simulink model "Y3Tiltrotor_sim3_IINDI"  (R2025a)
settings: Solver=ode4  StartTime=0.0  StopTime=60  FixedStep=uavParam.sampleTime  RelTol=1e-3
PreLoadFcn:
  | filepath  = fileparts(get_param(bdroot, 'FileName'))
  | cd(filepath);
InitFcn:
  | Init_sim_IINDI;
values from neighbouring files (symbols this model uses):
  a_HOD_p = 5    [Init_sim_IINDI.m]
  a_HOD_q = 5    [Init_sim_IINDI.m]
  a_HOD_r = 5    [Init_sim_IINDI.m]
  a_HOD_u = 5    [Init_sim_IINDI.m]
  a_HOD_v = 2    [Init_sim_IINDI.m]
  a_HOD_w = 30    [Init_sim_IINDI.m]
  control = struct    [Init_sim_IINDI.m]
  env = struct    [InitData.m]
  flightState = struct    [Init_sim_IINDI.m]
  FWSpeed0 = 15    [Init_sim_IINDI.m]
  k_lpf_p = 50    [Init_sim_IINDI.m]
  k_lpf_q = 80    [Init_sim_IINDI.m]
  k_lpf_r = 100    [Init_sim_IINDI.m]
  k_lpf_u = 10    [Init_sim_IINDI.m]
  k_lpf_v = 1.5    [Init_sim_IINDI.m]
  k_lpf_w = 50    [Init_sim_IINDI.m]
  k_p = 5    [Init_sim_IINDI.m]
  k_q = 12    [Init_sim_IINDI.m]
  k_r = 0.1    [Init_sim_IINDI.m]
  k_u = 1    [Init_sim_IINDI.m]
  k_v = 0.7    [Init_sim_IINDI.m]
  k_w = 2    [Init_sim_IINDI.m]
  l_p = 30    [Init_sim_IINDI.m]
  l_q = 15    [Init_sim_IINDI.m]
  l_r = 25    [Init_sim_IINDI.m]
  l_u = 10    [Init_sim_IINDI.m]
  l_v = 1.2    [Init_sim_IINDI.m]
  l_w = 1    [Init_sim_IINDI.m]
  lamda_p = 10    [Init_sim_IINDI.m]
  lamda_q = 5    [Init_sim_IINDI.m]
  lamda_r = 1    [Init_sim_IINDI.m]
  lamda_u = 1    [Init_sim_IINDI.m]
  lamda_v = 0.15    [Init_sim_IINDI.m]
  lamda_w = 1    [Init_sim_IINDI.m]
  uavParam = struct    [InitData.m]
undefined symbols (not defined in the file or in its folder): a_HOD, a_HOD_uvw, ControlSampleTime, F, Light, MIL, Newton, Raphson
libraries: slpidlib x30, SignalEditorBlockLib x13, simulink x3, aerolibtransform2 x3, sharedtransform x3, robotcorelib x3, matrix_library x3, aerolibasang x2, aerolibutil x2, aerolibwind2 x2, shared6dof x1, aerolibatmos2 x1
(part 5 of 7)

== system Y3Tiltrotor_sim3_IINDI/Subsystem/固定翼模态/高度-速度控制/定速模式/airspeed control ==
  Manual : Inport
  Airspeed_d : Inport  Port=2
  V_ref : Inport  Port=3
  Airspeed : Inport  Port=4
  PID Controller1 : slpidlib/PID Controller  Controller=PID  Form=Parallel  TimeDomain=Continuous-time  UseExternalTs=off  SampleTime=ControlSampleTime  IntegratorMethod=Forward Euler  FilterMethod=Forward Euler  ControllerParametersSource=internal  P=control.FW.airspeed_P  I=control.FW.airspeed_I  UseKiTs=off  D=control.FW.airspeed_D  UseExternalDerivativeSource=off  N=100  UseFilter=on  TunerSelectOption=Transfer Function Based (PID Tuner App)  InitialConditionSource=internal  InitialConditionForIntegrator=0  InitialConditionForFilter=0  DifferentiatorICPrevScaledInput=0  ExternalReset=none  TrackingMode=off  Kt=1  LimitOutput=on  SatLimitsSource=internal  UpperSaturationLimit=1  LowerSaturationLimit=0  LinearizeAsGain=on  AntiWindupMode=clamping  Kb=1  LimitIntegrator=off  UpperIntegratorSaturationLimit=inf  LowerIntegratorSaturationLimit=-inf  POutMin=[]  POutMax=[]  IOutMin=[]  IOutMax=[]  DOutMin=[]  DOutMax=[]  NOutMin=[]  NOutMax=[]  SumOutMin=[]  SumOutMax=[]  SaturationOutMin=[]  SaturationOutMax=[]  PParamMin=[]  PParamMax=[]  IParamMin=[]  IParamMax=[]  DParamMin=[]  DParamMax=[]  NParamMin=[]  NParamMax=[]  KbParamMin=[]  KbParamMax=[]  KtParamMin=[]  KtParamMax=[]  KbOutMin=[]  KbOutMax=[]  KtOutMin=[]  KtOutMax=[]  IntegratorOutMin=[]  IntegratorOutMax=[]  FilterOutMin=[]  FilterOutMax=[]  SumI1OutMin=[]  SumI1OutMax=[]  SumI2OutMin=[]  SumI2OutMax=[]  SumI3OutMin=[]  SumI3OutMax=[]  SumI4OutMin=[]  SumI4OutMax=[]  SumDOutMin=[]  SumDOutMax=[]  DifferentiatorOutMin=[]  DifferentiatorOutMax=[]  FilterDiffOutCoefMin=[]  FilterDiffOutCoefMax=[]  ReciprocalOutMin=[]  ReciprocalOutMax=[]  SumDenOutMin=[]  SumDenOutMax=[]  SumNumOutMin=[]  SumNumOutMax=[]  DivideOutMin=[]  DivideOutMax=[]  UdiffTsProdOutMin=[]  UdiffTsProdOutMax=[]  NTsProdOutMin=[]  NTsProdOutMax=[]  UintegralTsProdOutMin=[]  UintegralTsProdOutMax=[]  UngainTsProdOutMin=[]  UngainTsProdOutMax=[]  ClampingZeroOutDataTypeStr=Inherit: Inherit via back propagation  ClampingZeroOutMin=[]  ClampingZeroOutMax=[]  FilterDenConstantOutDataTypeStr=Inherit: Inherit via back propagation  FilterDenConstantOutMin=[]  FilterDenConstantOutMax=[]  PCopyOutDataTypeStr=Inherit: Inherit via back propagation  PCopyOutMin=[]  PCopyOutMax=[]  NCopyOutDataTypeStr=Inherit: Inherit via back propagation  NCopyOutMin=[]  NCopyOutMax=[]  IntegratorContinuousStateAttributes=''  IntegratorStateMustResolveToSignalObject=off  IntegratorRTWStateStorageClass=Auto  FilterContinuousStateAttributes=''  FilterStateMustResolveToSignalObject=off  FilterRTWStateStorageClass=Auto  ParallelPVariant=InternalParameters  IdealPVariant=Disabled  IVariant=InternalParameters  DVariant=InternalParameters  IntegratorVariant=Continuous  SatVariant=Enabled  AWVariant=ContClampingParallel  PCopyVariant=Disabled  TRVariant=Disabled  FdbkBlocksVariant=Forward  IdealPFdbkVariant=Disabled  SatFdbkVariant=Disabled  DerivativeFilterVariant=ContFilter  NVariant=InternalParameters  NCopyVariant=Disabled  FilterICVariant=InternalICsFilter  IntegratorICVariant=InternalICs  ExternalResetVariant=Disabled  TRSumVariant=Passthrough  SumFdbkVariant=Disabled  SumVariant=Sum_PID  TsampFilterVariant=InternalTs  TsampNgainVariant=Passthrough  TsampIntegralVariant=Disabled_SignalSpec  ExternalSaturationOutDataTypeStr=Inherit: Same as second input  DerivativeSourceVariant=ErrorSignal  PreIntVariant=InternalPreInt
  Sum : Sum  Inputs=|+-
  Switch : Switch  Criteria=u2 > Threshold  SaturateOnIntegerOverflow=off  InputSameDT=off
  Throttle : Outport
  wires:
  Sum/1 -> PID Controller1/1
  Airspeed/1 -> Sum/2
  PID Controller1/1 -> Throttle/1
  Switch/1 -> Sum/1
  Manual/1 -> Switch/2
  Airspeed_d/1 -> Switch/1
  V_ref/1 -> Switch/3

== system Y3Tiltrotor_sim3_IINDI/Subsystem/固定翼模态/高度-速度控制/定高模式/Subsystem ==
  Manual : Inport
  Height_d : Inport  Port=2
  Manual Vz_d : Inport  Port=3
  Xe : Inport  Port=4
  InputConditioning_altitude : Subsystem
  Merge : Merge
  Subsystem : Subsystem
  Switch Case : SwitchCase  CaseConditions={0,1}  ShowDefaultCase=off
  Vz_d : Outport
  wires:
  Manual/1 -> Switch Case/1
  Xe/1 -> Subsystem/2(Xe), InputConditioning_altitude/2(Xe)
  Subsystem/1(PID_vz_cmd) -> Merge/1  "PID vz_d"
  InputConditioning_altitude/1(manual_vz_cmd) -> Merge/2  "Manual vz_d"
  Merge/1 -> Vz_d/1
  Switch Case/1 -> Subsystem/Action
  Switch Case/2 -> InputConditioning_altitude/Action
  Manual Vz_d/1 -> InputConditioning_altitude/1(Manual Vz_d)
  Height_d/1 -> Subsystem/1(Navigation Z)

== system Y3Tiltrotor_sim3_IINDI/Subsystem/多旋翼模态/Multirotor XY control/Subsystem/InputConditioning_altitude ==
  Ch2 : Inport
  Action Port : ActionPort  ActionPortLabel=case [ 1 ]:
  Saturation1 : Saturate  UpperLimit=1  LowerLimit=-1
  deadzone3 : MATLAB Function  TreatAsAtomicUnit=on
  max_vy : Gain  Gain=control.maxMRvelocity_lat  OutDataTypeStr=Inherit: Inherit via back propagation
  manual_vlat_cmd : Outport  VectorParamsAs1DForOutWhenUnconnected=off
  wires:
  Ch2/1 -> deadzone3/1(u)
  deadzone3/1(y) -> Saturation1/1
  Saturation1/1 -> max_vy/1
  max_vy/1 -> manual_vlat_cmd/1

== system Y3Tiltrotor_sim3_IINDI/Subsystem/多旋翼模态/Multirotor XY control/Subsystem/Subsystem ==
  y_ref : Inport
  y : Inport  Port=2
  Action Port : ActionPort  ActionPortLabel=case [ 0 ]:
  Derivative : Derivative
  Saturation : Saturate  UpperLimit=control.maxMRvelocity_lat  LowerLimit=-control.maxMRvelocity_lat
  Sum : Sum  Inputs=|+-
  Sum1 : Sum  Inputs=++|
  Transfer Fcn1 : TransferFcn  Numerator=[5]  Denominator=[1 5]
  Transfer Fcn7 : TransferFcn  Numerator=[10]  Denominator=[1 10]
  Y position controller : slpidlib/PID Controller  Controller=PID  Form=Parallel  TimeDomain=Continuous-time  UseExternalTs=off  SampleTime=-1  IntegratorMethod=Forward Euler  FilterMethod=Forward Euler  ControllerParametersSource=internal  P=control.MR.y_P  I=control.MR.y_I  UseKiTs=off  D=control.MR.y_D  UseExternalDerivativeSource=off  N=100  UseFilter=on  TunerSelectOption=Transfer Function Based (PID Tuner App)  InitialConditionSource=internal  InitialConditionForIntegrator=0  InitialConditionForFilter=0  DifferentiatorICPrevScaledInput=0  ExternalReset=none  TrackingMode=off  Kt=1  LimitOutput=off  SatLimitsSource=internal  UpperSaturationLimit=control.maxMRvelocity_lat  LowerSaturationLimit=-control.maxMRvelocity_lat  LinearizeAsGain=on  AntiWindupMode=clamping  Kb=1  LimitIntegrator=off  UpperIntegratorSaturationLimit=inf  LowerIntegratorSaturationLimit=-inf  POutMin=[]  POutMax=[]  IOutMin=[]  IOutMax=[]  DOutMin=[]  DOutMax=[]  NOutMin=[]  NOutMax=[]  SumOutMin=[]  SumOutMax=[]  SaturationOutMin=[]  SaturationOutMax=[]  PParamMin=[]  PParamMax=[]  IParamMin=[]  IParamMax=[]  DParamMin=[]  DParamMax=[]  NParamMin=[]  NParamMax=[]  KbParamMin=[]  KbParamMax=[]  KtParamMin=[]  KtParamMax=[]  KbOutMin=[]  KbOutMax=[]  KtOutMin=[]  KtOutMax=[]  IntegratorOutMin=[]  IntegratorOutMax=[]  FilterOutMin=[]  FilterOutMax=[]  SumI1OutMin=[]  SumI1OutMax=[]  SumI2OutMin=[]  SumI2OutMax=[]  SumI3OutMin=[]  SumI3OutMax=[]  SumI4OutMin=[]  SumI4OutMax=[]  SumDOutMin=[]  SumDOutMax=[]  DifferentiatorOutMin=[]  DifferentiatorOutMax=[]  FilterDiffOutCoefMin=[]  FilterDiffOutCoefMax=[]  ReciprocalOutMin=[]  ReciprocalOutMax=[]  SumDenOutMin=[]  SumDenOutMax=[]  SumNumOutMin=[]  SumNumOutMax=[]  DivideOutMin=[]  DivideOutMax=[]  UdiffTsProdOutMin=[]  UdiffTsProdOutMax=[]  NTsProdOutMin=[]  NTsProdOutMax=[]  UintegralTsProdOutMin=[]  UintegralTsProdOutMax=[]  UngainTsProdOutMin=[]  UngainTsProdOutMax=[]  ClampingZeroOutDataTypeStr=Inherit: Inherit via back propagation  ClampingZeroOutMin=[]  ClampingZeroOutMax=[]  FilterDenConstantOutDataTypeStr=Inherit: Inherit via back propagation  FilterDenConstantOutMin=[]  FilterDenConstantOutMax=[]  PCopyOutDataTypeStr=Inherit: Inherit via back propagation  PCopyOutMin=[]  PCopyOutMax=[]  NCopyOutDataTypeStr=Inherit: Inherit via back propagation  NCopyOutMin=[]  NCopyOutMax=[]  IntegratorContinuousStateAttributes=''  IntegratorStateMustResolveToSignalObject=off  IntegratorRTWStateStorageClass=Auto  FilterContinuousStateAttributes=''  FilterStateMustResolveToSignalObject=off  FilterRTWStateStorageClass=Auto  ParallelPVariant=InternalParameters  IdealPVariant=Disabled  IVariant=InternalParameters  DVariant=InternalParameters  IntegratorVariant=Continuous  SatVariant=Disabled  AWVariant=Passthrough  PCopyVariant=Disabled  TRVariant=Disabled  FdbkBlocksVariant=Forward  IdealPFdbkVariant=Disabled  SatFdbkVariant=Disabled  DerivativeFilterVariant=ContFilter  NVariant=InternalParameters  NCopyVariant=Disabled  FilterICVariant=InternalICsFilter  IntegratorICVariant=InternalICs  ExternalResetVariant=Disabled  TRSumVariant=Passthrough  SumFdbkVariant=Disabled  SumVariant=Sum_PID  TsampFilterVariant=InternalTs  TsampNgainVariant=Passthrough  TsampIntegralVariant=Disabled_SignalSpec  ExternalSaturationOutDataTypeStr=Inherit: Same as second input  DerivativeSourceVariant=ErrorSignal  PreIntVariant=InternalPreInt
  PID_vy_cmd : Outport
  wires:
  y_ref/1 -> Transfer Fcn1/1
  y/1 -> Sum/2
  Sum/1 -> Y position controller/1  "e_y_IINDI"
  Saturation/1 -> PID_vy_cmd/1
  Sum1/1 -> Saturation/1
  Y position controller/1 -> Sum1/2
  Derivative/1 -> Transfer Fcn7/1
  Transfer Fcn7/1 -> Sum1/1
  Transfer Fcn1/1 -> Derivative/1, Sum/1  "y_ref"

== system Y3Tiltrotor_sim3_IINDI/Subsystem/多旋翼模态/Multirotor XY control/Subsystem3/InputConditioning_altitude ==
  Ch8 : Inport
  Action Port : ActionPort  ActionPortLabel=case [ 1 ]:
  Saturation1 : Saturate  UpperLimit=1  LowerLimit=-1
  deadzone3 : MATLAB Function  TreatAsAtomicUnit=on
  max_vx : Gain  Gain=control.maxMRvelocity_for  OutDataTypeStr=Inherit: Inherit via back propagation
  vx_d : SignalEditorBlockLib/Signal Editor  FileName=vx_d.mat  ActiveScenario=Test  ActiveSignal=定点-前向速度测试-遥控器  IsBus=off  OutputBusObjectStr=Bus: BusObject  SampleTime=0  ZeroCross=off  OutputAfterFinalValue=Setting to zero  Unit=inherit  PreserveSignalName=on  ApplySigPropsToAllScenarios=on  ApplySigPropsToAllSignals=off  SignalPropertySource=Dialog parameters
  manual_vfor_cmd : Outport  VectorParamsAs1DForOutWhenUnconnected=off
  wires:
  Saturation1/1 -> max_vx/1
  deadzone3/1(y) -> Saturation1/1
  Ch8/1 -> deadzone3/1(u)
  max_vx/1 -> manual_vfor_cmd/1

== system Y3Tiltrotor_sim3_IINDI/Subsystem/多旋翼模态/Multirotor XY control/Subsystem3/Subsystem ==
  x_ref : Inport
  x : Inport  Port=2
  Action Port : ActionPort  ActionPortLabel=case [ 0 ]:
  Derivative : Derivative
  Saturation : Saturate  UpperLimit=control.maxMRvelocity_for  LowerLimit=-control.maxMRvelocity_back
  Sum : Sum  Inputs=|+-
  Sum1 : Sum  Inputs=++|
  Transfer Fcn1 : TransferFcn  Numerator=[5]  Denominator=[1 5]
  Transfer Fcn7 : TransferFcn  Numerator=[10]  Denominator=[1 10]
  X position controller : slpidlib/PID Controller  Controller=PID  Form=Parallel  TimeDomain=Continuous-time  UseExternalTs=off  SampleTime=-1  IntegratorMethod=Forward Euler  FilterMethod=Forward Euler  ControllerParametersSource=internal  P=control.MR.x_P  I=control.MR.x_I  UseKiTs=off  D=control.MR.x_D  UseExternalDerivativeSource=off  N=5  UseFilter=on  TunerSelectOption=Transfer Function Based (PID Tuner App)  InitialConditionSource=internal  InitialConditionForIntegrator=0  InitialConditionForFilter=0  DifferentiatorICPrevScaledInput=0  ExternalReset=none  TrackingMode=off  Kt=1  LimitOutput=off  SatLimitsSource=internal  UpperSaturationLimit=control.maxMRvelocity_for  LowerSaturationLimit=-control.maxMRvelocity_back  LinearizeAsGain=on  AntiWindupMode=none  Kb=1  LimitIntegrator=off  UpperIntegratorSaturationLimit=inf  LowerIntegratorSaturationLimit=-inf  POutMin=[]  POutMax=[]  IOutMin=[]  IOutMax=[]  DOutMin=[]  DOutMax=[]  NOutMin=[]  NOutMax=[]  SumOutMin=[]  SumOutMax=[]  SaturationOutMin=[]  SaturationOutMax=[]  PParamMin=[]  PParamMax=[]  IParamMin=[]  IParamMax=[]  DParamMin=[]  DParamMax=[]  NParamMin=[]  NParamMax=[]  KbParamMin=[]  KbParamMax=[]  KtParamMin=[]  KtParamMax=[]  KbOutMin=[]  KbOutMax=[]  KtOutMin=[]  KtOutMax=[]  IntegratorOutMin=[]  IntegratorOutMax=[]  FilterOutMin=[]  FilterOutMax=[]  SumI1OutMin=[]  SumI1OutMax=[]  SumI2OutMin=[]  SumI2OutMax=[]  SumI3OutMin=[]  SumI3OutMax=[]  SumI4OutMin=[]  SumI4OutMax=[]  SumDOutMin=[]  SumDOutMax=[]  DifferentiatorOutMin=[]  DifferentiatorOutMax=[]  FilterDiffOutCoefMin=[]  FilterDiffOutCoefMax=[]  ReciprocalOutMin=[]  ReciprocalOutMax=[]  SumDenOutMin=[]  SumDenOutMax=[]  SumNumOutMin=[]  SumNumOutMax=[]  DivideOutMin=[]  DivideOutMax=[]  UdiffTsProdOutMin=[]  UdiffTsProdOutMax=[]  NTsProdOutMin=[]  NTsProdOutMax=[]  UintegralTsProdOutMin=[]  UintegralTsProdOutMax=[]  UngainTsProdOutMin=[]  UngainTsProdOutMax=[]  ClampingZeroOutDataTypeStr=Inherit: Inherit via back propagation  ClampingZeroOutMin=[]  ClampingZeroOutMax=[]  FilterDenConstantOutDataTypeStr=Inherit: Inherit via back propagation  FilterDenConstantOutMin=[]  FilterDenConstantOutMax=[]  PCopyOutDataTypeStr=Inherit: Inherit via back propagation  PCopyOutMin=[]  PCopyOutMax=[]  NCopyOutDataTypeStr=Inherit: Inherit via back propagation  NCopyOutMin=[]  NCopyOutMax=[]  IntegratorContinuousStateAttributes=''  IntegratorStateMustResolveToSignalObject=off  IntegratorRTWStateStorageClass=Auto  FilterContinuousStateAttributes=''  FilterStateMustResolveToSignalObject=off  FilterRTWStateStorageClass=Auto  ParallelPVariant=InternalParameters  IdealPVariant=Disabled  IVariant=InternalParameters  DVariant=InternalParameters  IntegratorVariant=Continuous  SatVariant=Disabled  AWVariant=Passthrough  PCopyVariant=Disabled  TRVariant=Disabled  FdbkBlocksVariant=Forward  IdealPFdbkVariant=Disabled  SatFdbkVariant=Disabled  DerivativeFilterVariant=ContFilter  NVariant=InternalParameters  NCopyVariant=Disabled  FilterICVariant=InternalICsFilter  IntegratorICVariant=InternalICs  ExternalResetVariant=Disabled  TRSumVariant=Passthrough  SumFdbkVariant=Disabled  SumVariant=Sum_PID  TsampFilterVariant=InternalTs  TsampNgainVariant=Passthrough  TsampIntegralVariant=Disabled_SignalSpec  ExternalSaturationOutDataTypeStr=Inherit: Same as second input  DerivativeSourceVariant=ErrorSignal  PreIntVariant=InternalPreInt
  PID_vx_cmd : Outport
  wires:
  x/1 -> Sum/2
  x_ref/1 -> Transfer Fcn1/1
  Sum/1 -> X position controller/1  "e_x_IINDI"
  Saturation/1 -> PID_vx_cmd/1
  X position controller/1 -> Sum1/2
  Sum1/1 -> Saturation/1
  Transfer Fcn7/1 -> Sum1/1
  Derivative/1 -> Transfer Fcn7/1
  Transfer Fcn1/1 -> Derivative/1, Sum/1  "x_ref"

== system Y3Tiltrotor_sim3_IINDI/Subsystem/多旋翼模态/Multirotor XY control1/Subsystem/InputConditioning_altitude ==
  Ch2 : Inport
  Action Port : ActionPort
  Saturation1 : Saturate  UpperLimit=1  LowerLimit=-1
  deadzone3 : MATLAB Function  TreatAsAtomicUnit=on
  max_vy : Gain  Gain=control.maxMRvelocity_lat  OutDataTypeStr=Inherit: Inherit via back propagation
  manual_vlat_cmd : Outport  VectorParamsAs1DForOutWhenUnconnected=off
  wires:
  Ch2/1 -> deadzone3/1(u)
  deadzone3/1(y) -> Saturation1/1
  Saturation1/1 -> max_vy/1
  max_vy/1 -> manual_vlat_cmd/1

== system Y3Tiltrotor_sim3_IINDI/Subsystem/多旋翼模态/Multirotor XY control1/Subsystem/Subsystem ==
  e_x : Inport
  e_y : Inport  Port=2
  e_z : Inport  Port=3
  DCMbe : Inport  Port=4
  Action Port : ActionPort
  Lateral position controller : slpidlib/PID Controller  Controller=PID  Form=Parallel  TimeDomain=Continuous-time  UseExternalTs=off  SampleTime=-1  IntegratorMethod=Forward Euler  FilterMethod=Forward Euler  ControllerParametersSource=internal  P=control.MR.y_P  I=control.MR.y_I  UseKiTs=off  D=control.MR.y_D  UseExternalDerivativeSource=off  N=100  UseFilter=on  TunerSelectOption=Transfer Function Based (PID Tuner App)  InitialConditionSource=internal  InitialConditionForIntegrator=0  InitialConditionForFilter=0  DifferentiatorICPrevScaledInput=0  ExternalReset=none  TrackingMode=off  Kt=1  LimitOutput=on  SatLimitsSource=internal  UpperSaturationLimit=control.maxMRvelocity_lat  LowerSaturationLimit=-control.maxMRvelocity_lat  LinearizeAsGain=on  AntiWindupMode=clamping  Kb=1  LimitIntegrator=off  UpperIntegratorSaturationLimit=inf  LowerIntegratorSaturationLimit=-inf  POutMin=[]  POutMax=[]  IOutMin=[]  IOutMax=[]  DOutMin=[]  DOutMax=[]  NOutMin=[]  NOutMax=[]  SumOutMin=[]  SumOutMax=[]  SaturationOutMin=[]  SaturationOutMax=[]  PParamMin=[]  PParamMax=[]  IParamMin=[]  IParamMax=[]  DParamMin=[]  DParamMax=[]  NParamMin=[]  NParamMax=[]  KbParamMin=[]  KbParamMax=[]  KtParamMin=[]  KtParamMax=[]  KbOutMin=[]  KbOutMax=[]  KtOutMin=[]  KtOutMax=[]  IntegratorOutMin=[]  IntegratorOutMax=[]  FilterOutMin=[]  FilterOutMax=[]  SumI1OutMin=[]  SumI1OutMax=[]  SumI2OutMin=[]  SumI2OutMax=[]  SumI3OutMin=[]  SumI3OutMax=[]  SumI4OutMin=[]  SumI4OutMax=[]  SumDOutMin=[]  SumDOutMax=[]  DifferentiatorOutMin=[]  DifferentiatorOutMax=[]  FilterDiffOutCoefMin=[]  FilterDiffOutCoefMax=[]  ReciprocalOutMin=[]  ReciprocalOutMax=[]  SumDenOutMin=[]  SumDenOutMax=[]  SumNumOutMin=[]  SumNumOutMax=[]  DivideOutMin=[]  DivideOutMax=[]  UdiffTsProdOutMin=[]  UdiffTsProdOutMax=[]  NTsProdOutMin=[]  NTsProdOutMax=[]  UintegralTsProdOutMin=[]  UintegralTsProdOutMax=[]  UngainTsProdOutMin=[]  UngainTsProdOutMax=[]  ClampingZeroOutDataTypeStr=Inherit: Inherit via back propagation  ClampingZeroOutMin=[]  ClampingZeroOutMax=[]  FilterDenConstantOutDataTypeStr=Inherit: Inherit via back propagation  FilterDenConstantOutMin=[]  FilterDenConstantOutMax=[]  PCopyOutDataTypeStr=Inherit: Inherit via back propagation  PCopyOutMin=[]  PCopyOutMax=[]  NCopyOutDataTypeStr=Inherit: Inherit via back propagation  NCopyOutMin=[]  NCopyOutMax=[]  IntegratorContinuousStateAttributes=''  IntegratorStateMustResolveToSignalObject=off  IntegratorRTWStateStorageClass=Auto  FilterContinuousStateAttributes=''  FilterStateMustResolveToSignalObject=off  FilterRTWStateStorageClass=Auto  ParallelPVariant=InternalParameters  IdealPVariant=Disabled  IVariant=InternalParameters  DVariant=InternalParameters  IntegratorVariant=Continuous  SatVariant=Enabled  AWVariant=ContClampingParallel  PCopyVariant=Disabled  TRVariant=Disabled  FdbkBlocksVariant=Forward  IdealPFdbkVariant=Disabled  SatFdbkVariant=Disabled  DerivativeFilterVariant=ContFilter  NVariant=InternalParameters  NCopyVariant=Disabled  FilterICVariant=InternalICsFilter  IntegratorICVariant=InternalICs  ExternalResetVariant=Disabled  TRSumVariant=Passthrough  SumFdbkVariant=Disabled  SumVariant=Sum_PID  TsampFilterVariant=InternalTs  TsampNgainVariant=Passthrough  TsampIntegralVariant=Disabled_SignalSpec  ExternalSaturationOutDataTypeStr=Inherit: Same as second input  DerivativeSourceVariant=ErrorSignal  PreIntVariant=InternalPreInt
  Mux : Mux  Inputs=3
  Product : Product  Multiplication=Matrix(*)
  Reshape : Reshape  OutputDimensionality=Column vector (2-D)
  Reshape1 : Reshape
  Selector : Selector  InputPortWidth=3  IndexOptions=Index vector (dialog)  Indices=[2]  OutputSizes=1
  PID_vlat_cmd : Outport
  wires:
  Selector/1 -> Lateral position controller/1  "MR_e_lat"
  DCMbe/1 -> Product/1
  e_x/1 -> Mux/1
  e_y/1 -> Mux/2
  e_z/1 -> Mux/3
  Mux/1 -> Reshape/1
  Reshape/1 -> Product/2
  Product/1 -> Reshape1/1
  Reshape1/1 -> Selector/1
  Lateral position controller/1 -> PID_vlat_cmd/1

== system Y3Tiltrotor_sim3_IINDI/Subsystem/多旋翼模态/Multirotor XY control1/Subsystem3/InputConditioning_altitude ==
  Ch8 : Inport
  Action Port : ActionPort
  Saturation1 : Saturate  UpperLimit=1  LowerLimit=-1
  deadzone3 : MATLAB Function  TreatAsAtomicUnit=on
  max_vx : Gain  Gain=control.maxMRvelocity_for  OutDataTypeStr=Inherit: Inherit via back propagation
  vx_d : SignalEditorBlockLib/Signal Editor  FileName=vx_d.mat  ActiveScenario=Test  ActiveSignal=定点-前向速度测试-遥控器  IsBus=off  OutputBusObjectStr=Bus: BusObject  SampleTime=0  ZeroCross=off  OutputAfterFinalValue=Setting to zero  Unit=inherit  PreserveSignalName=on  ApplySigPropsToAllScenarios=on  ApplySigPropsToAllSignals=off  SignalPropertySource=Dialog parameters
  manual_vfor_cmd : Outport  VectorParamsAs1DForOutWhenUnconnected=off
  wires:
  Saturation1/1 -> max_vx/1
  deadzone3/1(y) -> Saturation1/1
  Ch8/1 -> deadzone3/1(u)
  max_vx/1 -> manual_vfor_cmd/1

== system Y3Tiltrotor_sim3_IINDI/Subsystem/多旋翼模态/Multirotor XY control1/Subsystem3/Subsystem ==
  e_x : Inport
  e_y : Inport  Port=2
  e_z : Inport  Port=3
  DCMbe : Inport  Port=4
  Action Port : ActionPort
  Forward position controller : slpidlib/PID Controller  Controller=PID  Form=Parallel  TimeDomain=Continuous-time  UseExternalTs=off  SampleTime=-1  IntegratorMethod=Forward Euler  FilterMethod=Forward Euler  ControllerParametersSource=internal  P=control.MR.x_P  I=control.MR.x_I  UseKiTs=off  D=control.MR.x_D  UseExternalDerivativeSource=off  N=100  UseFilter=on  TunerSelectOption=Transfer Function Based (PID Tuner App)  InitialConditionSource=internal  InitialConditionForIntegrator=0  InitialConditionForFilter=0  DifferentiatorICPrevScaledInput=0  ExternalReset=none  TrackingMode=off  Kt=1  LimitOutput=on  SatLimitsSource=internal  UpperSaturationLimit=control.maxMRvelocity_for  LowerSaturationLimit=-control.maxMRvelocity_back  LinearizeAsGain=on  AntiWindupMode=none  Kb=1  LimitIntegrator=off  UpperIntegratorSaturationLimit=inf  LowerIntegratorSaturationLimit=-inf  POutMin=[]  POutMax=[]  IOutMin=[]  IOutMax=[]  DOutMin=[]  DOutMax=[]  NOutMin=[]  NOutMax=[]  SumOutMin=[]  SumOutMax=[]  SaturationOutMin=[]  SaturationOutMax=[]  PParamMin=[]  PParamMax=[]  IParamMin=[]  IParamMax=[]  DParamMin=[]  DParamMax=[]  NParamMin=[]  NParamMax=[]  KbParamMin=[]  KbParamMax=[]  KtParamMin=[]  KtParamMax=[]  KbOutMin=[]  KbOutMax=[]  KtOutMin=[]  KtOutMax=[]  IntegratorOutMin=[]  IntegratorOutMax=[]  FilterOutMin=[]  FilterOutMax=[]  SumI1OutMin=[]  SumI1OutMax=[]  SumI2OutMin=[]  SumI2OutMax=[]  SumI3OutMin=[]  SumI3OutMax=[]  SumI4OutMin=[]  SumI4OutMax=[]  SumDOutMin=[]  SumDOutMax=[]  DifferentiatorOutMin=[]  DifferentiatorOutMax=[]  FilterDiffOutCoefMin=[]  FilterDiffOutCoefMax=[]  ReciprocalOutMin=[]  ReciprocalOutMax=[]  SumDenOutMin=[]  SumDenOutMax=[]  SumNumOutMin=[]  SumNumOutMax=[]  DivideOutMin=[]  DivideOutMax=[]  UdiffTsProdOutMin=[]  UdiffTsProdOutMax=[]  NTsProdOutMin=[]  NTsProdOutMax=[]  UintegralTsProdOutMin=[]  UintegralTsProdOutMax=[]  UngainTsProdOutMin=[]  UngainTsProdOutMax=[]  ClampingZeroOutDataTypeStr=Inherit: Inherit via back propagation  ClampingZeroOutMin=[]  ClampingZeroOutMax=[]  FilterDenConstantOutDataTypeStr=Inherit: Inherit via back propagation  FilterDenConstantOutMin=[]  FilterDenConstantOutMax=[]  PCopyOutDataTypeStr=Inherit: Inherit via back propagation  PCopyOutMin=[]  PCopyOutMax=[]  NCopyOutDataTypeStr=Inherit: Inherit via back propagation  NCopyOutMin=[]  NCopyOutMax=[]  IntegratorContinuousStateAttributes=''  IntegratorStateMustResolveToSignalObject=off  IntegratorRTWStateStorageClass=Auto  FilterContinuousStateAttributes=''  FilterStateMustResolveToSignalObject=off  FilterRTWStateStorageClass=Auto  ParallelPVariant=InternalParameters  IdealPVariant=Disabled  IVariant=InternalParameters  DVariant=InternalParameters  IntegratorVariant=Continuous  SatVariant=Enabled  AWVariant=Passthrough  PCopyVariant=Disabled  TRVariant=Disabled  FdbkBlocksVariant=Forward  IdealPFdbkVariant=Disabled  SatFdbkVariant=Disabled  DerivativeFilterVariant=ContFilter  NVariant=InternalParameters  NCopyVariant=Disabled  FilterICVariant=InternalICsFilter  IntegratorICVariant=InternalICs  ExternalResetVariant=Disabled  TRSumVariant=Passthrough  SumFdbkVariant=Disabled  SumVariant=Sum_PID  TsampFilterVariant=InternalTs  TsampNgainVariant=Passthrough  TsampIntegralVariant=Disabled_SignalSpec  ExternalSaturationOutDataTypeStr=Inherit: Same as second input  DerivativeSourceVariant=ErrorSignal  PreIntVariant=InternalPreInt
  Mux : Mux  Inputs=3
  Product : Product  Multiplication=Matrix(*)
  Reshape : Reshape  OutputDimensionality=Column vector (2-D)
  Reshape1 : Reshape
  Selector : Selector  InputPortWidth=3  IndexOptions=Index vector (dialog)  Indices=[1]  OutputSizes=1
  PID_vfor_cmd : Outport
  wires:
  Forward position controller/1 -> PID_vfor_cmd/1
  Selector/1 -> Forward position controller/1  "MR_e_f"
  e_z/1 -> Mux/3
  Reshape1/1 -> Selector/1
  Reshape/1 -> Product/2
  e_y/1 -> Mux/2
  Mux/1 -> Reshape/1
  e_x/1 -> Mux/1
  DCMbe/1 -> Product/1
  Product/1 -> Reshape1/1

== system Y3Tiltrotor_sim3_IINDI/Subsystem/多旋翼模态/Multirotor altitude control/Subsystem/InputConditioning_altitude ==
  Ch3 : Inport
  Xe : Inport  Port=2
  Action Port : ActionPort  ActionPortLabel=case [ 1 ]:
  Constant1 : Constant  Value=1000
  Gain1 : Gain  Commented=on  Gain=1/1000
  MATLAB Function : MATLAB Function  TreatAsAtomicUnit=on
  Manual Switch : ManualSwitch  CurrentSetting=0
  PID Controller : slpidlib/PID Controller  Controller=PID  Form=Parallel  TimeDomain=Continuous-time  UseExternalTs=off  SampleTime=ControlSampleTime  IntegratorMethod=Forward Euler  FilterMethod=Forward Euler  ControllerParametersSource=internal  P=control.MR.alt_P  I=control.MR.alt_I  UseKiTs=off  D=control.MR.alt_D  UseExternalDerivativeSource=off  N=100  UseFilter=on  TunerSelectOption=Transfer Function Based (PID Tuner App)  InitialConditionSource=internal  InitialConditionForIntegrator=0  InitialConditionForFilter=0  DifferentiatorICPrevScaledInput=0  ExternalReset=none  TrackingMode=off  Kt=1  LimitOutput=on  SatLimitsSource=internal  UpperSaturationLimit=control.maxMRvelocity  LowerSaturationLimit=-control.maxMRvelocity  LinearizeAsGain=on  AntiWindupMode=clamping  Kb=1  LimitIntegrator=off  UpperIntegratorSaturationLimit=inf  LowerIntegratorSaturationLimit=-inf  POutMin=[]  POutMax=[]  IOutMin=[]  IOutMax=[]  DOutMin=[]  DOutMax=[]  NOutMin=[]  NOutMax=[]  SumOutMin=[]  SumOutMax=[]  SaturationOutMin=[]  SaturationOutMax=[]  PParamMin=[]  PParamMax=[]  IParamMin=[]  IParamMax=[]  DParamMin=[]  DParamMax=[]  NParamMin=[]  NParamMax=[]  KbParamMin=[]  KbParamMax=[]  KtParamMin=[]  KtParamMax=[]  KbOutMin=[]  KbOutMax=[]  KtOutMin=[]  KtOutMax=[]  IntegratorOutMin=[]  IntegratorOutMax=[]  FilterOutMin=[]  FilterOutMax=[]  SumI1OutMin=[]  SumI1OutMax=[]  SumI2OutMin=[]  SumI2OutMax=[]  SumI3OutMin=[]  SumI3OutMax=[]  SumI4OutMin=[]  SumI4OutMax=[]  SumDOutMin=[]  SumDOutMax=[]  DifferentiatorOutMin=[]  DifferentiatorOutMax=[]  FilterDiffOutCoefMin=[]  FilterDiffOutCoefMax=[]  ReciprocalOutMin=[]  ReciprocalOutMax=[]  SumDenOutMin=[]  SumDenOutMax=[]  SumNumOutMin=[]  SumNumOutMax=[]  DivideOutMin=[]  DivideOutMax=[]  UdiffTsProdOutMin=[]  UdiffTsProdOutMax=[]  NTsProdOutMin=[]  NTsProdOutMax=[]  UintegralTsProdOutMin=[]  UintegralTsProdOutMax=[]  UngainTsProdOutMin=[]  UngainTsProdOutMax=[]  ClampingZeroOutDataTypeStr=Inherit: Inherit via back propagation  ClampingZeroOutMin=[]  ClampingZeroOutMax=[]  FilterDenConstantOutDataTypeStr=Inherit: Inherit via back propagation  FilterDenConstantOutMin=[]  FilterDenConstantOutMax=[]  PCopyOutDataTypeStr=Inherit: Inherit via back propagation  PCopyOutMin=[]  PCopyOutMax=[]  NCopyOutDataTypeStr=Inherit: Inherit via back propagation  NCopyOutMin=[]  NCopyOutMax=[]  IntegratorContinuousStateAttributes=''  IntegratorStateMustResolveToSignalObject=off  IntegratorRTWStateStorageClass=Auto  FilterContinuousStateAttributes=''  FilterStateMustResolveToSignalObject=off  FilterRTWStateStorageClass=Auto  ParallelPVariant=InternalParameters  IdealPVariant=Disabled  IVariant=InternalParameters  DVariant=InternalParameters  IntegratorVariant=Continuous  SatVariant=Enabled  AWVariant=ContClampingParallel  PCopyVariant=Disabled  TRVariant=Disabled  FdbkBlocksVariant=Forward  IdealPFdbkVariant=Disabled  SatFdbkVariant=Disabled  DerivativeFilterVariant=ContFilter  NVariant=InternalParameters  NCopyVariant=Disabled  FilterICVariant=InternalICsFilter  IntegratorICVariant=InternalICs  ExternalResetVariant=Disabled  TRSumVariant=Passthrough  SumFdbkVariant=Disabled  SumVariant=Sum_PID  TsampFilterVariant=InternalTs  TsampNgainVariant=Passthrough  TsampIntegralVariant=Disabled_SignalSpec  ExternalSaturationOutDataTypeStr=Inherit: Same as second input  DerivativeSourceVariant=ErrorSignal  PreIntVariant=InternalPreInt
  Saturation1 : Saturate  UpperLimit=1  LowerLimit=-1
  Saturation10 : Saturate  Commented=on  UpperLimit=1  LowerLimit=0
  Selector : Selector  InputPortWidth=3  IndexOptions=Index vector (dialog)  Indices=3  OutputSizes=1
  Sum1 : Sum  Inputs=|+-
  Sum2 : Sum  Inputs=|+-
  Unary Minus : UnaryMinus
  deadzone3 : MATLAB Function  TreatAsAtomicUnit=on
  max_vz : Gain  Gain=control.maxMRvelocity  OutDataTypeStr=Inherit: Inherit via back propagation
  max_z : Gain  Commented=on  Gain=500  OutDataTypeStr=Inherit: Inherit via back propagation
  sim1_z_d : SignalEditorBlockLib/Signal Editor  FileName=vz_d.mat  ActiveScenario=Test  ActiveSignal=直接给定高度-遥控器  IsBus=off  OutputBusObjectStr=Bus: BusObject  SampleTime=0  ZeroCross=off  OutputAfterFinalValue=Setting to zero  Unit=inherit  PreserveSignalName=on  ApplySigPropsToAllScenarios=on  ApplySigPropsToAllSignals=on  SignalPropertySource=Dialog parameters
  Manual vz_d : Outport  VectorParamsAs1DForOutWhenUnconnected=off
  wires:
  deadzone3/1(y) -> Saturation1/1
  Xe/1 -> Selector/1
  Saturation10/1 -> max_z/1
  Unary Minus/1 -> Sum1/2
  Sum1/1 -> PID Controller/1
  ? -> Sum1/1  "manual_z_cmd"
  Selector/1 -> MATLAB Function/2(z_e), Unary Minus/1
  Constant1/1 -> Sum2/2
  Sum2/1 -> Gain1/1
  Gain1/1 -> Saturation10/1
  Ch3/1 -> deadzone3/1(u), Sum2/1
  Manual Switch/1 -> Manual vz_d/1
  PID Controller/1 -> Manual Switch/2
  Saturation1/1 -> max_vz/1
  max_vz/1 -> MATLAB Function/1(u)
  MATLAB Function/1(vz_cmd) -> Manual Switch/1

== system Y3Tiltrotor_sim3_IINDI/Subsystem/多旋翼模态/Multirotor altitude control/Subsystem/Subsystem ==
  z_ref : Inport
  z : Inport  Port=2
  Action Port : ActionPort  ActionPortLabel=case [ 0 ]:
  Derivative : Derivative
  PID Controller : slpidlib/PID Controller  Controller=PID  Form=Parallel  TimeDomain=Continuous-time  UseExternalTs=off  SampleTime=ControlSampleTime  IntegratorMethod=Forward Euler  FilterMethod=Forward Euler  ControllerParametersSource=internal  P=control.MR.alt_P  I=control.MR.alt_I  UseKiTs=off  D=control.MR.alt_D  UseExternalDerivativeSource=off  N=100  UseFilter=on  TunerSelectOption=Transfer Function Based (PID Tuner App)  InitialConditionSource=internal  InitialConditionForIntegrator=0  InitialConditionForFilter=0  DifferentiatorICPrevScaledInput=0  ExternalReset=none  TrackingMode=off  Kt=1  LimitOutput=off  SatLimitsSource=internal  UpperSaturationLimit=control.maxMRvelocity  LowerSaturationLimit=-control.maxMRvelocity  LinearizeAsGain=on  AntiWindupMode=clamping  Kb=1  LimitIntegrator=off  UpperIntegratorSaturationLimit=inf  LowerIntegratorSaturationLimit=-inf  POutMin=[]  POutMax=[]  IOutMin=[]  IOutMax=[]  DOutMin=[]  DOutMax=[]  NOutMin=[]  NOutMax=[]  SumOutMin=[]  SumOutMax=[]  SaturationOutMin=[]  SaturationOutMax=[]  PParamMin=[]  PParamMax=[]  IParamMin=[]  IParamMax=[]  DParamMin=[]  DParamMax=[]  NParamMin=[]  NParamMax=[]  KbParamMin=[]  KbParamMax=[]  KtParamMin=[]  KtParamMax=[]  KbOutMin=[]  KbOutMax=[]  KtOutMin=[]  KtOutMax=[]  IntegratorOutMin=[]  IntegratorOutMax=[]  FilterOutMin=[]  FilterOutMax=[]  SumI1OutMin=[]  SumI1OutMax=[]  SumI2OutMin=[]  SumI2OutMax=[]  SumI3OutMin=[]  SumI3OutMax=[]  SumI4OutMin=[]  SumI4OutMax=[]  SumDOutMin=[]  SumDOutMax=[]  DifferentiatorOutMin=[]  DifferentiatorOutMax=[]  FilterDiffOutCoefMin=[]  FilterDiffOutCoefMax=[]  ReciprocalOutMin=[]  ReciprocalOutMax=[]  SumDenOutMin=[]  SumDenOutMax=[]  SumNumOutMin=[]  SumNumOutMax=[]  DivideOutMin=[]  DivideOutMax=[]  UdiffTsProdOutMin=[]  UdiffTsProdOutMax=[]  NTsProdOutMin=[]  NTsProdOutMax=[]  UintegralTsProdOutMin=[]  UintegralTsProdOutMax=[]  UngainTsProdOutMin=[]  UngainTsProdOutMax=[]  ClampingZeroOutDataTypeStr=Inherit: Inherit via back propagation  ClampingZeroOutMin=[]  ClampingZeroOutMax=[]  FilterDenConstantOutDataTypeStr=Inherit: Inherit via back propagation  FilterDenConstantOutMin=[]  FilterDenConstantOutMax=[]  PCopyOutDataTypeStr=Inherit: Inherit via back propagation  PCopyOutMin=[]  PCopyOutMax=[]  NCopyOutDataTypeStr=Inherit: Inherit via back propagation  NCopyOutMin=[]  NCopyOutMax=[]  IntegratorContinuousStateAttributes=''  IntegratorStateMustResolveToSignalObject=off  IntegratorRTWStateStorageClass=Auto  FilterContinuousStateAttributes=''  FilterStateMustResolveToSignalObject=off  FilterRTWStateStorageClass=Auto  ParallelPVariant=InternalParameters  IdealPVariant=Disabled  IVariant=InternalParameters  DVariant=InternalParameters  IntegratorVariant=Continuous  SatVariant=Disabled  AWVariant=Passthrough  PCopyVariant=Disabled  TRVariant=Disabled  FdbkBlocksVariant=Forward  IdealPFdbkVariant=Disabled  SatFdbkVariant=Disabled  DerivativeFilterVariant=ContFilter  NVariant=InternalParameters  NCopyVariant=Disabled  FilterICVariant=InternalICsFilter  IntegratorICVariant=InternalICs  ExternalResetVariant=Disabled  TRSumVariant=Passthrough  SumFdbkVariant=Disabled  SumVariant=Sum_PID  TsampFilterVariant=InternalTs  TsampNgainVariant=Passthrough  TsampIntegralVariant=Disabled_SignalSpec  ExternalSaturationOutDataTypeStr=Inherit: Same as second input  DerivativeSourceVariant=ErrorSignal  PreIntVariant=InternalPreInt
  Saturation : Saturate  UpperLimit=control.maxMRvelocity  LowerLimit=-control.maxMRvelocity
  Sum : Sum  Inputs=|+-
  Sum1 : Sum  Inputs=++|
  Transfer Fcn1 : TransferFcn  Numerator=[5]  Denominator=[1 5]
  Transfer Fcn7 : TransferFcn  Numerator=[10]  Denominator=[1 10]
  PID_vz_cmd : Outport
  wires:
  z_ref/1 -> Transfer Fcn1/1
  z/1 -> Sum/2
  Sum/1 -> PID Controller/1  "e_z_IINDI"
  PID Controller/1 -> Sum1/2
  Derivative/1 -> Transfer Fcn7/1
  Sum1/1 -> Saturation/1
  Saturation/1 -> PID_vz_cmd/1
  Transfer Fcn7/1 -> Sum1/1
  Transfer Fcn1/1 -> Derivative/1, Sum/1  "z_ref"

== system Y3Tiltrotor_sim3_IINDI/Subsystem/多旋翼模态/Multirotor attitude control (IINDI)/INDI in vector form/Subsystem ==
  original : Inport
  Demux : Demux  Outputs=3
  Mux : Mux  Inputs=3
  Transfer Fcn1 : TransferFcn  Numerator=[k_lpf_q]  Denominator=[1 k_lpf_q]
  Transfer Fcn2 : TransferFcn  Numerator=[k_lpf_r]  Denominator=[1 k_lpf_r]
  Transfer Fcn3 : TransferFcn  Numerator=[k_lpf_p]  Denominator=[1 k_lpf_p]
  LPF : Outport
  wires:
  Demux/2 -> Transfer Fcn1/1
  Demux/1 -> Transfer Fcn3/1
  Mux/1 -> LPF/1
  Transfer Fcn3/1 -> Mux/1
  Transfer Fcn1/1 -> Mux/2
  Transfer Fcn2/1 -> Mux/3
  Demux/3 -> Transfer Fcn2/1
  original/1 -> Demux/1

== system Y3Tiltrotor_sim3_IINDI/Subsystem/多旋翼模态/Multirotor attitude control (IINDI)/INDI in vector form/Subsystem1 ==
  original : Inport
  Demux : Demux  Outputs=3
  Mux : Mux  Inputs=3
  Transfer Fcn1 : TransferFcn  Numerator=[k_lpf_q]  Denominator=[1 k_lpf_q]
  Transfer Fcn2 : TransferFcn  Numerator=[k_lpf_r]  Denominator=[1 k_lpf_r]
  Transfer Fcn3 : TransferFcn  Numerator=[k_lpf_p]  Denominator=[1 k_lpf_p]
  LPF : Outport
  wires:
  Demux/2 -> Transfer Fcn1/1
  Demux/1 -> Transfer Fcn3/1
  Mux/1 -> LPF/1
  Transfer Fcn3/1 -> Mux/1
  Transfer Fcn1/1 -> Mux/2
  Transfer Fcn2/1 -> Mux/3
  Demux/3 -> Transfer Fcn2/1
  original/1 -> Demux/1

== system Y3Tiltrotor_sim3_IINDI/Subsystem/多旋翼模态/Multirotor attitude control (IINDI)/INDI in vector form/Subsystem2 ==
  original : Inport
  Demux : Demux  Outputs=3
  Mux : Mux  Inputs=3
  Transfer Fcn1 : TransferFcn  Numerator=[k_lpf_q]  Denominator=[1 k_lpf_q]
  Transfer Fcn2 : TransferFcn  Numerator=[k_lpf_r]  Denominator=[1 k_lpf_r]
  Transfer Fcn3 : TransferFcn  Numerator=[k_lpf_p]  Denominator=[1 k_lpf_p]
  LPF : Outport
  wires:
  Demux/2 -> Transfer Fcn1/1
  Demux/1 -> Transfer Fcn3/1
  Mux/1 -> LPF/1
  Transfer Fcn3/1 -> Mux/1
  Transfer Fcn1/1 -> Mux/2
  Transfer Fcn2/1 -> Mux/3
  Demux/3 -> Transfer Fcn2/1
  original/1 -> Demux/1

== system Y3Tiltrotor_sim3_IINDI/Subsystem/多旋翼模态/Multirotor attitude control (IINDI)/Improved INDI in vector form/6阶HOD ==
  X1 : Inport
  Gain : Gain  Gain=[4*a_HOD_p^2 0 0;0 4*a_HOD_q^2 0;0 0 4*a_HOD_r^2]  Multiplication=Matrix(K*u) (u vector)
  Gain1 : Gain  Gain=[4*a_HOD_p 0 0;0 4*a_HOD_q 0;0 0 4*a_HOD_r]  Multiplication=Matrix(K*u) (u vector)
  Integrator : Integrator  InitialCondition=[0 0 0]'
  Integrator1 : Integrator  InitialCondition=[0 0 0]'
  Sum : Sum  Inputs=|+-
  Sum1 : Sum  Inputs=++|
  X1_dot_hat : Outport
  wires:
  Gain1/1 -> Sum1/1
  Integrator1/1 -> Sum1/2  "x2_hat"
  Gain/1 -> Integrator1/1
  Sum1/1 -> Integrator/1, X1_dot_hat/1
  Sum/1 -> Gain1/1, Gain/1
  X1/1 -> Sum/1
  Integrator/1 -> Sum/2  "x1_hat"

== system Y3Tiltrotor_sim3_IINDI/Subsystem/多旋翼模态/Multirotor attitude control (IINDI)/Improved INDI in vector form/6阶HOD1 ==
  X1 : Inport
  Gain : Gain  Gain=[4*a_HOD_p^2 0 0;0 4*a_HOD_q^2 0;0 0 4*a_HOD_r^2]  Multiplication=Matrix(K*u) (u vector)
  Gain1 : Gain  Gain=[4*a_HOD_p 0 0;0 4*a_HOD_q 0;0 0 4*a_HOD_r]  Multiplication=Matrix(K*u) (u vector)
  Integrator : Integrator  InitialCondition=[0 0 0]'
  Integrator1 : Integrator  InitialCondition=[0 0 0]'
  Sum : Sum  Inputs=|+-
  Sum1 : Sum  Inputs=++|
  X1_dot_hat : Outport
  wires:
  Integrator/1 -> Sum/2  "x1_hat"
  X1/1 -> Sum/1
  Sum/1 -> Gain/1, Gain1/1
  Sum1/1 -> X1_dot_hat/1, Integrator/1
  Gain/1 -> Integrator1/1
  Integrator1/1 -> Sum1/2  "x2_hat"
  Gain1/1 -> Sum1/1

== system Y3Tiltrotor_sim3_IINDI/Subsystem/多旋翼模态/Multirotor attitude control (IINDI)/Improved INDI in vector form/CFO ==
  x1_dot : Inport
  x1 : Inport  Port=2
  bu : Inport  Port=3
  Gain : Gain  Gain=[l_p 0 0;0 l_q 0;0 0 l_r]  Multiplication=Matrix(K*u) (u vector)
  Gain1 : Gain  Gain=[lamda_p 0 0;0 lamda_q 0;0 0 lamda_r]  Multiplication=Matrix(K*u) (u vector)
  Integrator : Integrator  InitialCondition=[0 0 0]'
  Integrator1 : Integrator  InitialCondition=[0 0 0]'
  Sum : Sum  Inputs=|+-
  Sum1 : Sum  Inputs=+++
  Sum2 : Sum  Inputs=++|
  d_hat : Outport
  wires:
  Sum2/1 -> d_hat/1, Sum1/1
  Integrator1/1 -> Sum2/2  "x2_hat"
  Gain1/1 -> Integrator1/1
  Sum/1 -> Gain/1
  Gain/1 -> Gain1/1, Sum2/1
  bu/1 -> Sum1/3
  x1_dot/1 -> Sum1/2
  Sum1/1 -> Integrator/1
  Integrator/1 -> Sum/2  "x1_hat"
  x1/1 -> Sum/1

== system Y3Tiltrotor_sim3_IINDI/Subsystem/多旋翼模态/Multirotor attitude control (IINDI)/Improved INDI in vector form/Subsystem ==
  original : Inport
  Demux : Demux  Outputs=3
  Mux : Mux  Inputs=3
  Transfer Fcn1 : TransferFcn  Numerator=[k_lpf_q]  Denominator=[1 k_lpf_q]
  Transfer Fcn2 : TransferFcn  Numerator=[k_lpf_r]  Denominator=[1 k_lpf_r]
  Transfer Fcn3 : TransferFcn  Numerator=[k_lpf_p]  Denominator=[1 k_lpf_p]
  LPF : Outport
  wires:
  Demux/2 -> Transfer Fcn1/1
  Demux/1 -> Transfer Fcn3/1
  Mux/1 -> LPF/1
  Transfer Fcn3/1 -> Mux/1
  Transfer Fcn1/1 -> Mux/2
  Transfer Fcn2/1 -> Mux/3
  Demux/3 -> Transfer Fcn2/1
  original/1 -> Demux/1

== system Y3Tiltrotor_sim3_IINDI/Subsystem/多旋翼模态/Multirotor attitude control (IINDI)/Improved INDI in vector form/Subsystem2 ==
  original : Inport
  Demux : Demux  Outputs=3
  Mux : Mux  Inputs=3
  Transfer Fcn1 : TransferFcn  Numerator=[k_lpf_q]  Denominator=[1 k_lpf_q]
  Transfer Fcn2 : TransferFcn  Numerator=[k_lpf_r]  Denominator=[1 k_lpf_r]
  Transfer Fcn3 : TransferFcn  Numerator=[k_lpf_p]  Denominator=[1 k_lpf_p]
  LPF : Outport
  wires:
  Demux/2 -> Transfer Fcn1/1
  Demux/1 -> Transfer Fcn3/1
  Mux/1 -> LPF/1
  Transfer Fcn3/1 -> Mux/1
  Transfer Fcn1/1 -> Mux/2
  Transfer Fcn2/1 -> Mux/3
  Demux/3 -> Transfer Fcn2/1
  original/1 -> Demux/1

== system Y3Tiltrotor_sim3_IINDI/Subsystem/多旋翼模态/Multirotor attitude control (IINDI)/Improved INDI_p/2阶HOD ==
  X1 : Inport
  Gain : Gain  Gain=4*a_HOD^2
  Gain1 : Gain  Gain=4*a_HOD
  Integrator : Integrator
  Integrator1 : Integrator
  Sum : Sum  Inputs=|+-
  Sum1 : Sum  Inputs=++|
  X1_dot_hat : Outport
  wires:
  Gain1/1 -> Sum1/1
  Integrator1/1 -> Sum1/2  "x2_hat"
  Gain/1 -> Integrator1/1
  Sum1/1 -> Integrator/1, X1_dot_hat/1
  Sum/1 -> Gain1/1, Gain/1
  X1/1 -> Sum/1
  Integrator/1 -> Sum/2  "x1_hat"

== system Y3Tiltrotor_sim3_IINDI/Subsystem/多旋翼模态/Multirotor attitude control (IINDI)/Improved INDI_p/CFO ==
  x1_dot : Inport
  x1 : Inport  Port=2
  bu : Inport  Port=3
  Gain : Gain  Gain=l_p
  Gain1 : Gain  Gain=lamda_p
  Integrator : Integrator
  Integrator1 : Integrator
  Sum : Sum  Inputs=|+-
  Sum1 : Sum  Inputs=+++
  Sum2 : Sum  Inputs=++|
  d_hat : Outport
  wires:
  Sum2/1 -> d_hat/1, Sum1/1
  Integrator1/1 -> Sum2/2  "x2_hat"
  Gain1/1 -> Integrator1/1
  Sum/1 -> Gain/1
  Gain/1 -> Gain1/1, Sum2/1
  bu/1 -> Sum1/3
  x1_dot/1 -> Sum1/2
  Sum1/1 -> Integrator/1
  Integrator/1 -> Sum/2  "x1_hat"
  x1/1 -> Sum/1

== system Y3Tiltrotor_sim3_IINDI/Subsystem/多旋翼模态/Multirotor attitude control (IINDI)/Improved INDI_q/2阶HOD ==
  X1 : Inport
  Gain : Gain  Gain=4*a_HOD^2
  Gain1 : Gain  Gain=4*a_HOD
  Integrator : Integrator
  Integrator1 : Integrator
  Sum : Sum  Inputs=|+-
  Sum1 : Sum  Inputs=++|
  X1_dot_hat : Outport
  wires:
  Integrator/1 -> Sum/2  "x1_hat"
  X1/1 -> Sum/1
  Sum/1 -> Gain/1, Gain1/1
  Sum1/1 -> X1_dot_hat/1, Integrator/1
  Gain/1 -> Integrator1/1
  Integrator1/1 -> Sum1/2  "x2_hat"
  Gain1/1 -> Sum1/1

== system Y3Tiltrotor_sim3_IINDI/Subsystem/多旋翼模态/Multirotor attitude control (IINDI)/Improved INDI_q/CFO ==
  x1_dot : Inport
  x1 : Inport  Port=2
  bu : Inport  Port=3
  Gain : Gain  Gain=l_q
  Gain1 : Gain  Gain=lamda_q
  Integrator : Integrator
  Integrator1 : Integrator
  Sum : Sum  Inputs=|+-
  Sum1 : Sum  Inputs=+++
  Sum2 : Sum  Inputs=++|
  d_hat : Outport
  wires:
  x1/1 -> Sum/1
  Integrator/1 -> Sum/2  "x1_hat"
  Sum1/1 -> Integrator/1
  x1_dot/1 -> Sum1/2
  bu/1 -> Sum1/3
  Gain/1 -> Sum2/1, Gain1/1
  Sum/1 -> Gain/1
  Gain1/1 -> Integrator1/1
  Integrator1/1 -> Sum2/2  "x2_hat"
  Sum2/1 -> Sum1/1, d_hat/1

== system Y3Tiltrotor_sim3_IINDI/Subsystem/多旋翼模态/Multirotor attitude control (IINDI)/Improved INDI_r/2阶HOD ==
  X1 : Inport
  Gain : Gain  Gain=4*a_HOD^2
  Gain1 : Gain  Gain=4*a_HOD
  Integrator : Integrator
  Integrator1 : Integrator
  Sum : Sum  Inputs=|+-
  Sum1 : Sum  Inputs=++|
  X1_dot_hat : Outport
  wires:
  Gain1/1 -> Sum1/1
  Integrator1/1 -> Sum1/2  "x2_hat"
  Gain/1 -> Integrator1/1
  Sum1/1 -> Integrator/1, X1_dot_hat/1
  Sum/1 -> Gain1/1, Gain/1
  X1/1 -> Sum/1
  Integrator/1 -> Sum/2  "x1_hat"

== system Y3Tiltrotor_sim3_IINDI/Subsystem/多旋翼模态/Multirotor attitude control (IINDI)/Improved INDI_r/CFO ==
  x1_dot : Inport
  x1 : Inport  Port=2
  bu : Inport  Port=3
  Gain : Gain  Gain=l_r
  Gain1 : Gain  Gain=lamda_r
  Integrator : Integrator
  Integrator1 : Integrator
  Sum : Sum  Inputs=|+-
  Sum1 : Sum  Inputs=+++
  Sum2 : Sum  Inputs=++|
  d_hat : Outport
  wires:
  Sum2/1 -> d_hat/1, Sum1/1
  Integrator1/1 -> Sum2/2  "x2_hat"
  Gain1/1 -> Integrator1/1
  Sum/1 -> Gain/1
  Gain/1 -> Gain1/1, Sum2/1
  bu/1 -> Sum1/3
  x1_dot/1 -> Sum1/2
  Sum1/1 -> Integrator/1
  Integrator/1 -> Sum/2  "x1_hat"
  x1/1 -> Sum/1

== system Y3Tiltrotor_sim3_IINDI/Subsystem/多旋翼模态/Multirotor attitude control (IINDI)/Subsystem/Subsystem ==
  Euler_d : Inport
  Euler : Inport  Port=2
  Action Port : ActionPort  ActionPortLabel=case [ 0 ]:
  Gain1 : Gain  Gain=pi/180
  PID Controller4 : slpidlib/PID Controller  Controller=PI  Form=Parallel  TimeDomain=Continuous-time  UseExternalTs=off  SampleTime=ControlSampleTime  IntegratorMethod=Forward Euler  FilterMethod=Forward Euler  ControllerParametersSource=internal  P=control.MR.yaw_P  I=control.MR.yaw_I  UseKiTs=off  D=0  UseExternalDerivativeSource=off  N=100  UseFilter=on  TunerSelectOption=Transfer Function Based (PID Tuner App)  InitialConditionSource=internal  InitialConditionForIntegrator=0  InitialConditionForFilter=0  DifferentiatorICPrevScaledInput=0  ExternalReset=none  TrackingMode=off  Kt=1  LimitOutput=on  SatLimitsSource=internal  UpperSaturationLimit=control.maxRollRate  LowerSaturationLimit=control.minRollRate  LinearizeAsGain=on  AntiWindupMode=clamping  Kb=1  LimitIntegrator=off  UpperIntegratorSaturationLimit=inf  LowerIntegratorSaturationLimit=-inf  POutMin=[]  POutMax=[]  IOutMin=[]  IOutMax=[]  DOutMin=[]  DOutMax=[]  NOutMin=[]  NOutMax=[]  SumOutMin=[]  SumOutMax=[]  SaturationOutMin=[]  SaturationOutMax=[]  PParamMin=[]  PParamMax=[]  IParamMin=[]  IParamMax=[]  DParamMin=[]  DParamMax=[]  NParamMin=[]  NParamMax=[]  KbParamMin=[]  KbParamMax=[]  KtParamMin=[]  KtParamMax=[]  KbOutMin=[]  KbOutMax=[]  KtOutMin=[]  KtOutMax=[]  IntegratorOutMin=[]  IntegratorOutMax=[]  FilterOutMin=[]  FilterOutMax=[]  SumI1OutMin=[]  SumI1OutMax=[]  SumI2OutMin=[]  SumI2OutMax=[]  SumI3OutMin=[]  SumI3OutMax=[]  SumI4OutMin=[]  SumI4OutMax=[]  SumDOutMin=[]  SumDOutMax=[]  DifferentiatorOutMin=[]  DifferentiatorOutMax=[]  FilterDiffOutCoefMin=[]  FilterDiffOutCoefMax=[]  ReciprocalOutMin=[]  ReciprocalOutMax=[]  SumDenOutMin=[]  SumDenOutMax=[]  SumNumOutMin=[]  SumNumOutMax=[]  DivideOutMin=[]  DivideOutMax=[]  UdiffTsProdOutMin=[]  UdiffTsProdOutMax=[]  NTsProdOutMin=[]  NTsProdOutMax=[]  UintegralTsProdOutMin=[]  UintegralTsProdOutMax=[]  UngainTsProdOutMin=[]  UngainTsProdOutMax=[]  ClampingZeroOutDataTypeStr=Inherit: Inherit via back propagation  ClampingZeroOutMin=[]  ClampingZeroOutMax=[]  FilterDenConstantOutDataTypeStr=Inherit: Inherit via back propagation  FilterDenConstantOutMin=[]  FilterDenConstantOutMax=[]  PCopyOutDataTypeStr=Inherit: Inherit via back propagation  PCopyOutMin=[]  PCopyOutMax=[]  NCopyOutDataTypeStr=Inherit: Inherit via back propagation  NCopyOutMin=[]  NCopyOutMax=[]  IntegratorContinuousStateAttributes=''  IntegratorStateMustResolveToSignalObject=off  IntegratorRTWStateStorageClass=Auto  FilterContinuousStateAttributes=''  FilterStateMustResolveToSignalObject=off  FilterRTWStateStorageClass=Auto  ParallelPVariant=InternalParameters  IdealPVariant=Disabled  IVariant=InternalParameters  DVariant=Disabled  IntegratorVariant=Continuous  SatVariant=Enabled  AWVariant=ContClampingParallel  PCopyVariant=Disabled  TRVariant=Disabled  FdbkBlocksVariant=Forward  IdealPFdbkVariant=Disabled  SatFdbkVariant=Disabled  DerivativeFilterVariant=Disabled  NVariant=Disabled  NCopyVariant=Disabled_SignalSpec  FilterICVariant=Disabled  IntegratorICVariant=InternalICs  ExternalResetVariant=Disabled  TRSumVariant=Passthrough  SumFdbkVariant=Disabled  SumVariant=Sum_PI  TsampFilterVariant=InternalTs  TsampNgainVariant=Passthrough  TsampIntegralVariant=Disabled_SignalSpec  ExternalSaturationOutDataTypeStr=Inherit: Same as second input  DerivativeSourceVariant=Disabled  PreIntVariant=InternalPreInt
  Selector4 : Selector  InputPortWidth=3  IndexOptions=Index vector (dialog)  Indices=3  OutputSizes=1
  Selector8 : Selector  InputPortWidth=3  IndexOptions=Index vector (dialog)  Indices=3  OutputSizes=1
  Sum4 : Sum  Inputs=|+-
  Transfer Fcn2 : TransferFcn  Numerator=[5]  Denominator=[1 5]
  MR_r_d : Outport
  wires:
  Euler/1 -> Selector8/1
  Gain1/1 -> Transfer Fcn2/1
  Selector4/1 -> Gain1/1
  Transfer Fcn2/1 -> Sum4/1
  Selector8/1 -> Sum4/2
  PID Controller4/1 -> MR_r_d/1
  Sum4/1 -> PID Controller4/1  "e_yaw_IINDI"
  Euler_d/1 -> Selector4/1
